simulink model "peltier_lazo_P"  (R2026a)
settings: Solver=ode23t  StartTime=0  StopTime=t_final  MaxStep=0.2  RelTol=1e-6  AbsTol=1e-8
values from neighbouring files (symbols this model uses):
  I0 = 1.19014918446    [parametros.mat]    (also in parametros_control.mat; peltier_modelo.m = fzero(@(I) [1 0]*equilibrio(I, p) - Tb_obj, [0, 2]); sensibilidad_P.m = fzero(@(i) temperatura_fria(i,p)-(10+273.15),[0 2]); sensibilidad_compensado.m = fzero(@(i) temperatura_fria(i,p)-(10+273.15),[0 2]))
  Imax = 2.0    (= 2)    [editar_ensayos.m]    (also in parametros_ensayos.mat)
  Imin = 0    [editar_ensayos.m]    (also in parametros_ensayos.mat)
  instante_ref = t_ref    [configurar.m]    (also in sensibilidad_P.m; sensibilidad_compensado.m; simular_P.m)
  Kp = Kp_base    [configurar.m]    (also in diseno_compensador.m = Kp_lista(i); sensibilidad_P.m; sensibilidad_compensado.m; simular_P.m = Kp_lista(k))
  p =     [parametros.mat]    (also in sensibilidad_P.m = p_nom; sensibilidad_compensado.m = p_nom; simular_P.m = p_nom)
  tau_corriente = 0.01    [editar_ensayos.m]    (also in parametros_ensayos.mat)
  Tc_init = Tc0    [configurar.m]    (also in sensibilidad_P.m; sensibilidad_compensado.m; simular_P.m = p.Tamb)
  Th_init = Th0    [configurar.m]    (also in sensibilidad_P.m; sensibilidad_compensado.m; simular_P.m = p.Tamb)
libraries: fl_lib x28, nesl_utility x10
Description:
  | GR09 - P. e=Tb_medida-ref; mando=sat(I0+Kp*e,0,2); tau*dI/dt=mando-I.
settings Model: Creator=charl  LastModifiedBy=charl
settings DebuggingCC: AlgebraicLoopMsg=error

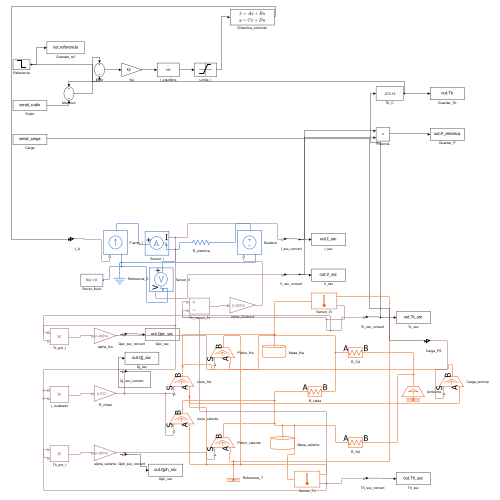
[thumbnail: Simulink's stored preview of the top-level diagram]
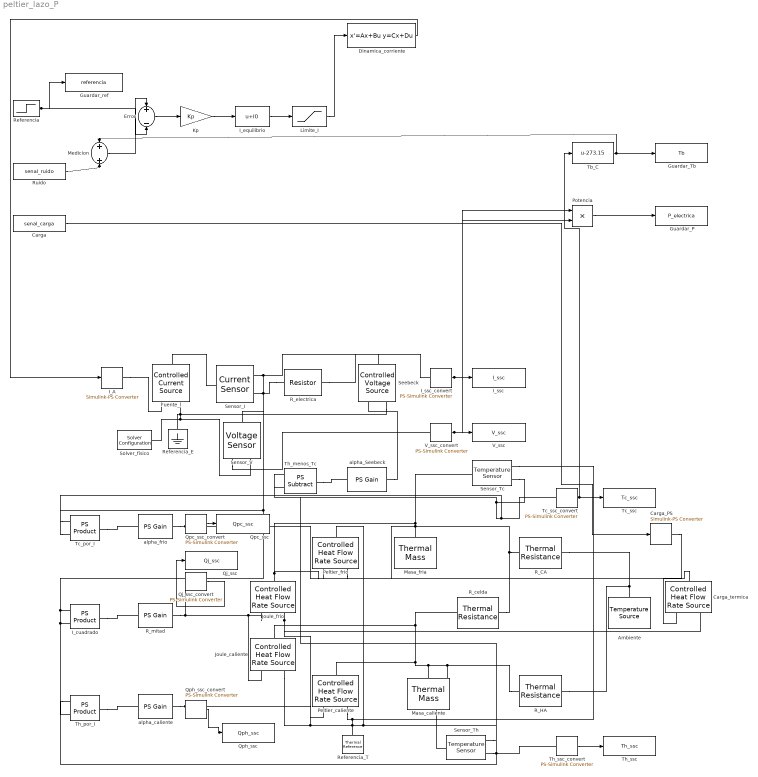
== system peltier_lazo_P ==
  Ambiente : fl_lib/Thermal/Thermal Sources/Temperature Source  temperature=p.Tamb K
  Carga : FromWorkspace  VariableName=senal_carga  Interpolate=off  OutputAfterFinalValue=Holding final value
  Carga_PS : nesl_utility/Simulink-PS Converter  PhysicalDomain=network_engine_domain  SubClassName=ps_input  LeftPortType=input  RightPortType=output  PseudoPeriodic=off  Frequencies=[]  NoiseDistribution=none  NoiseParameters=[]  Unit=W  AffineConversion=off  FilteringAndDerivatives=provide  SimscapeFilterOrder=1  InputFilterTimeConstant=0.001  UdotUserProvided=0
  Carga_termica : fl_lib/Thermal/Thermal Sources/Controlled Heat Flow Rate Source
  Dinamica_corriente : StateSpace  A=-1/tau_corriente  B=1/tau_corriente  D=0  InitialCondition=I0
  Error : Sum  Inputs=+-
  Fuente_I : fl_lib/Electrical/Electrical Sources/Controlled Current Source
  Guardar_P : ToWorkspace  VariableName=P_electrica  SaveFormat=Timeseries  SampleTime=-1
  Guardar_Tb : ToWorkspace  VariableName=Tb  SaveFormat=Timeseries  SampleTime=-1
  Guardar_ref : ToWorkspace  VariableName=referencia  SaveFormat=Timeseries  SampleTime=-1
  I_A : nesl_utility/Simulink-PS Converter  PhysicalDomain=network_engine_domain  SubClassName=ps_input  LeftPortType=input  RightPortType=output  PseudoPeriodic=off  Frequencies=[]  NoiseDistribution=none  NoiseParameters=[]  Unit=A  AffineConversion=off  FilteringAndDerivatives=provide  SimscapeFilterOrder=1  InputFilterTimeConstant=0.001  UdotUserProvided=0
  I_cuadrado : fl_lib/Physical Signals/Functions/PS Product
  I_equilibrio : Bias  Bias=I0  SaturateOnIntegerOverflow=off
  I_ssc : ToWorkspace  VariableName=I_ssc  SaveFormat=Timeseries  SampleTime=-1
  I_ssc_convert : nesl_utility/PS-Simulink Converter  PhysicalDomain=network_engine_domain  SubClassName=ps_output  LeftPortType=input  RightPortType=output  PseudoPeriodic=off  Frequencies=[]  VectorFormat=inherit  Unit=A  AffineConversion=off
  Joule_caliente : fl_lib/Thermal/Thermal Sources/Controlled Heat Flow Rate Source
  Joule_frio : fl_lib/Thermal/Thermal Sources/Controlled Heat Flow Rate Source
  Kp : Gain  Gain=Kp
  Limite_I : Saturate  UpperLimit=Imax  LowerLimit=Imin
  Masa_caliente : fl_lib/Thermal/Thermal Elements/Thermal Mass  mass_type=foundation.enum.constant_variable.constant  mass=p.mH kg  sp_heat=900 J/(kg*K)  mass_min=1e-6 kg  num_ports=foundation.enum.numPorts2.one  m_specify=off  m_priority=High  m=1 kg  m_nominal_specify=off  m_nominal_value=1  m_nominal_unit=kg  T_specify=on  T_priority=High  T=Th_init K  T_nominal_specify=off  T_nominal_value=1  T_nominal_unit=K  Q_specify=off  Q_priority=None  Q=0 W  Q_nominal_specify=off  Q_nominal_value=1  Q_nominal_unit=W
  Masa_fria : fl_lib/Thermal/Thermal Elements/Thermal Mass  mass_type=foundation.enum.constant_variable.constant  mass=p.mC kg  sp_heat=900 J/(kg*K)  mass_min=1e-6 kg  num_ports=foundation.enum.numPorts2.one  m_specify=off  m_priority=High  m=1 kg  m_nominal_specify=off  m_nominal_value=1  m_nominal_unit=kg  T_specify=on  T_priority=High  T=Tc_init K  T_nominal_specify=off  T_nominal_value=1  T_nominal_unit=K  Q_specify=off  Q_priority=None  Q=0 W  Q_nominal_specify=off  Q_nominal_value=1  Q_nominal_unit=W
  Medicion : Sum
  Peltier_caliente : fl_lib/Thermal/Thermal Sources/Controlled Heat Flow Rate Source
  Peltier_frio : fl_lib/Thermal/Thermal Sources/Controlled Heat Flow Rate Source
  Potencia : Product
  Qj_ssc : ToWorkspace  VariableName=Qj_ssc  SaveFormat=Timeseries  SampleTime=-1
  Qj_ssc_convert : nesl_utility/PS-Simulink Converter  PhysicalDomain=network_engine_domain  SubClassName=ps_output  LeftPortType=input  RightPortType=output  PseudoPeriodic=off  Frequencies=[]  VectorFormat=inherit  Unit=W  AffineConversion=off
  Qpc_ssc : ToWorkspace  VariableName=Qpc_ssc  SaveFormat=Timeseries  SampleTime=-1
  Qpc_ssc_convert : nesl_utility/PS-Simulink Converter  PhysicalDomain=network_engine_domain  SubClassName=ps_output  LeftPortType=input  RightPortType=output  PseudoPeriodic=off  Frequencies=[]  VectorFormat=inherit  Unit=W  AffineConversion=off
  Qph_ssc : ToWorkspace  VariableName=Qph_ssc  SaveFormat=Timeseries  SampleTime=-1
  Qph_ssc_convert : nesl_utility/PS-Simulink Converter  PhysicalDomain=network_engine_domain  SubClassName=ps_output  LeftPortType=input  RightPortType=output  PseudoPeriodic=off  Frequencies=[]  VectorFormat=inherit  Unit=W  AffineConversion=off
  R_CA : fl_lib/Thermal/Thermal Elements/Thermal Resistance  resistance=p.RCA K/W  T_specify=off  T_priority=None  T=0 K  T_nominal_specify=off  T_nominal_value=1  T_nominal_unit=K  Q_specify=off  Q_priority=None  Q=0 W  Q_nominal_specify=off  Q_nominal_value=1  Q_nominal_unit=W
  R_HA : fl_lib/Thermal/Thermal Elements/Thermal Resistance  resistance=case_RHA K/W  T_specify=off  T_priority=None  T=0 K  T_nominal_specify=off  T_nominal_value=1  T_nominal_unit=K  Q_specify=off  Q_priority=None  Q=0 W  Q_nominal_specify=off  Q_nominal_value=1  Q_nominal_unit=W
  R_celda : fl_lib/Thermal/Thermal Elements/Thermal Resistance  resistance=1/p.K K/W  T_specify=off  T_priority=None  T=0 K  T_nominal_specify=off  T_nominal_value=1  T_nominal_unit=K  Q_specify=off  Q_priority=None  Q=0 W  Q_nominal_specify=off  Q_nominal_value=1  Q_nominal_unit=W
  R_electrica : fl_lib/Electrical/Electrical Elements/Resistor  R=p.R Ohm  i_specify=off  i_priority=None  i=0 A  i_nominal_specify=off  i_nominal_value=1  i_nominal_unit=A  v_specify=off  v_priority=None  v=0 V  v_nominal_specify=off  v_nominal_value=1  v_nominal_unit=V
  R_mitad : fl_lib/Physical Signals/Functions/PS Gain  gain=p.R/2 Ohm
  Referencia : Step  Time=instante_ref  InitialValue=r_antes  FinalValue=r_despues  SampleTime=0
  Referencia_E : fl_lib/Electrical/Electrical Elements/Electrical Reference
  Referencia_T : fl_lib/Thermal/Thermal Elements/Thermal Reference
  Ruido : FromWorkspace  VariableName=senal_ruido  Interpolate=off  OutputAfterFinalValue=Holding final value
  Seebeck : fl_lib/Electrical/Electrical Sources/Controlled Voltage Source
  Sensor_I : fl_lib/Electrical/Electrical Sensors/Current Sensor
  Sensor_Tc : fl_lib/Thermal/Thermal Sensors/Temperature Sensor  temperature_measure=foundation.enum.MeasurementReference.difference
  Sensor_Th : fl_lib/Thermal/Thermal Sensors/Temperature Sensor  temperature_measure=foundation.enum.MeasurementReference.difference
  Sensor_V : fl_lib/Electrical/Electrical Sensors/Voltage Sensor
  Solver_fisico : nesl_utility/Solver Configuration  PhysicalDomain=network_engine_domain  SubClassName=solver  LeftPortType=input  RightPortType=generic  Tones=[]  Harmonics=[]  SimulateNoise=off  Profile=off  UseLocalSampling=off  EnableSwitchedLinearOptims=on  FrequencyDomain=off  UseCCode=off  RelTol=0.001  AbsTol=0.001  MinStep=1e-09  ToWorkspace=off  RevertToSquareIcSolve=off  NumHomotopyIterations=100  PhasorMode=off  PhasorModeNumHarmonics=1  ConsistencySolver=NEWTON_XTOL_AFTER_FTOL  CanonicalOrdering=UNORDERED  OptimizeIntermediates=UNOPTIMIZED  IndexReductionMethod=DerivativeReplacement  DoDC=off  ResidualTolerance=1e-09  ConsistencyTolSource=GLOBAL  ConsistencyAbsTol=0.001  ConsistencyRelTol=0.001  ConsistencyTolFactor=0.001  UseLocalSolver=off  LocalSolverChoice=NE_BACKWARD_EULER_ADVANCER  ResolveIndetEquations=on  FunctionEvalNumThread=1  LocalSolverSampleTime=0.001  DoFixedCost=off  MaxNonlinIter=3  MaxModeIter=2  ComputeImpulses=off  ImpulseIterations=2  LinearAlgebra=auto  LinearAlgebraNumThread=0  EquationFormulation=NE_TIME_EF  DelaysMemoryBudget=1024  AutomaticFiltering=on  FilteringTimeConstant=0.001  PartitionStorageMethod=AS_NEEDED  PartitionMemoryBudget=1024  PartitionMethod=ROBUST  MultibodyUseLocalSolver=off  MultibodyLocalSolverChoice=ODE1  MultibodyLocalSolverSampleTime=0.001
  Tb_C : Bias  Bias=-273.15  SaturateOnIntegerOverflow=off
  Tc_por_I : fl_lib/Physical Signals/Functions/PS Product
  Tc_ssc : ToWorkspace  VariableName=Tc_ssc  SaveFormat=Timeseries  SampleTime=-1
  Tc_ssc_convert : nesl_utility/PS-Simulink Converter  PhysicalDomain=network_engine_domain  SubClassName=ps_output  LeftPortType=input  RightPortType=output  PseudoPeriodic=off  Frequencies=[]  VectorFormat=inherit  Unit=K  AffineConversion=off
  Th_menos_Tc : fl_lib/Physical Signals/Functions/PS Subtract
  Th_por_I : fl_lib/Physical Signals/Functions/PS Product
  Th_ssc : ToWorkspace  VariableName=Th_ssc  SaveFormat=Timeseries  SampleTime=-1
  Th_ssc_convert : nesl_utility/PS-Simulink Converter  PhysicalDomain=network_engine_domain  SubClassName=ps_output  LeftPortType=input  RightPortType=output  PseudoPeriodic=off  Frequencies=[]  VectorFormat=inherit  Unit=K  AffineConversion=off
  V_ssc : ToWorkspace  VariableName=V_ssc  SaveFormat=Timeseries  SampleTime=-1
  V_ssc_convert : nesl_utility/PS-Simulink Converter  PhysicalDomain=network_engine_domain  SubClassName=ps_output  LeftPortType=input  RightPortType=output  PseudoPeriodic=off  Frequencies=[]  VectorFormat=inherit  Unit=V  AffineConversion=off
  alpha_Seebeck : fl_lib/Physical Signals/Functions/PS Gain  gain=p.alpha V/K
  alpha_caliente : fl_lib/Physical Signals/Functions/PS Gain  gain=p.alpha V/K
  alpha_frio : fl_lib/Physical Signals/Functions/PS Gain  gain=p.alpha V/K
  wires:
  Tc_ssc_convert/1 -> Tc_ssc/1, Tb_C/1
  Th_ssc_convert/1 -> Th_ssc/1
  I_ssc_convert/1 -> I_ssc/1, Potencia/2
  V_ssc_convert/1 -> V_ssc/1, Potencia/1
  Qpc_ssc_convert/1 -> Qpc_ssc/1
  Qph_ssc_convert/1 -> Qph_ssc/1
  Qj_ssc_convert/1 -> Qj_ssc/1
  Ruido/1 -> Medicion/2
  Tb_C/1 -> Medicion/1, Guardar_Tb/1
  Medicion/1 -> Error/1
  Referencia/1 -> Error/2, Guardar_ref/1
  Error/1 -> Kp/1
  Kp/1 -> I_equilibrio/1
  I_equilibrio/1 -> Limite_I/1
  Limite_I/1 -> Dinamica_corriente/1
  Potencia/1 -> Guardar_P/1
  Dinamica_corriente/1 -> I_A/1
  Carga/1 -> Carga_PS/1
  connections:
  I_A/RConn1 -- Fuente_I/RConn1
  Fuente_I/LConn1 -- Sensor_I/LConn1
  R_electrica/LConn1 -- Sensor_I/RConn2 -- Sensor_V/LConn1
  R_electrica/RConn1 -- Seebeck/LConn1
  Seebeck/RConn2 -- Sensor_V/RConn2 -- Solver_fisico/RConn1 -- Fuente_I/RConn2 -- Referencia_E/LConn1
  R_CA/LConn1 -- Masa_fria/LConn1 -- Sensor_Tc/LConn1 -- Joule_frio/LConn1 -- Carga_termica/LConn1 -- Peltier_frio/RConn2 -- R_celda/RConn1
  R_HA/LConn1 -- Joule_caliente/LConn1 -- R_celda/LConn1 -- Peltier_caliente/LConn1 -- Masa_caliente/LConn1 -- Sensor_Th/LConn1
  R_CA/RConn1 -- Ambiente/LConn1 -- R_HA/RConn1
  Sensor_Tc/RConn1 -- Peltier_frio/LConn1 -- Sensor_Th/RConn1 -- Joule_caliente/RConn2 -- Joule_frio/RConn2 -- Carga_termica/RConn2 -- Referencia_T/LConn1 -- Peltier_caliente/RConn2
  Tc_por_I/LConn1 -- Sensor_Tc/RConn2 -- Th_menos_Tc/LConn2 -- Tc_ssc_convert/LConn1
  Th_por_I/LConn1 -- Sensor_Th/RConn2 -- Th_menos_Tc/LConn1 -- Th_ssc_convert/LConn1
  Tc_por_I/LConn2 -- Th_por_I/LConn2 -- I_cuadrado/LConn2 -- I_cuadrado/LConn1 -- Sensor_I/RConn1 -- I_ssc_convert/LConn1
  Tc_por_I/RConn1 -- alpha_frio/LConn1
  Th_por_I/RConn1 -- alpha_caliente/LConn1
  I_cuadrado/RConn1 -- R_mitad/LConn1
  Peltier_frio/RConn1 -- alpha_frio/RConn1 -- Qpc_ssc_convert/LConn1
  Peltier_caliente/RConn1 -- alpha_caliente/RConn1 -- Qph_ssc_convert/LConn1
  Joule_frio/RConn1 -- R_mitad/RConn1 -- Qj_ssc_convert/LConn1 -- Joule_caliente/RConn1
  Th_menos_Tc/RConn1 -- alpha_Seebeck/LConn1
  alpha_Seebeck/RConn1 -- Seebeck/RConn1
  Sensor_V/RConn1 -- V_ssc_convert/LConn1
  Carga_PS/RConn1 -- Carga_termica/RConn1
